simulink model "RRTMS_Activity_State"  (R2026a)
settings: Solver=FixedStepDiscrete  StopTime=10  FixedStep=1
settings Model: Creator=HP  LastModifiedBy=HP

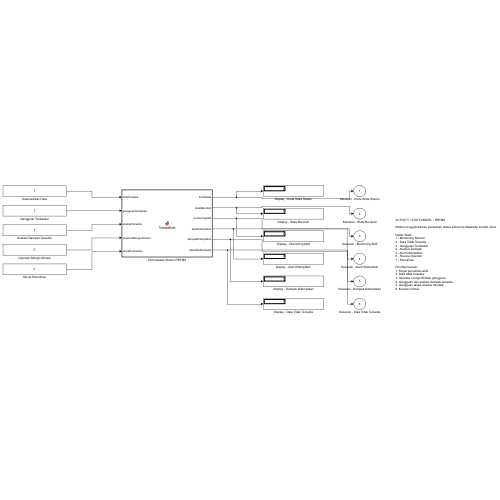
[thumbnail: Simulink's stored preview of the top-level diagram]
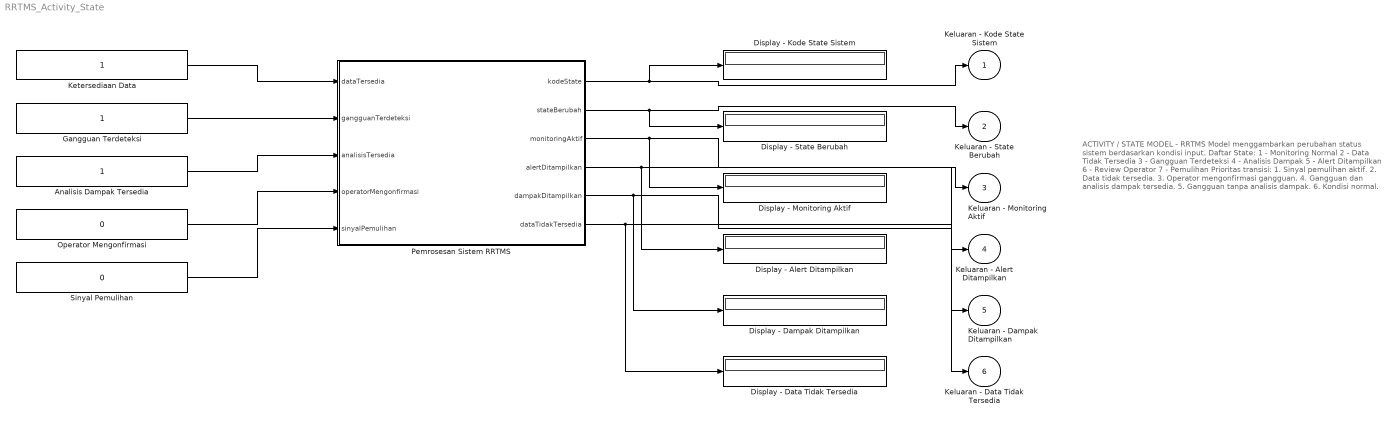
== system RRTMS_Activity_State ==
  note: ACTIVITY / STATE MODEL - RRTMS
      |
      | Model menggambarkan perubahan status sistem berdasarkan kondisi input.
      |
      | Daftar State:
      | 1 - Monitoring Normal
      | 2 - Data Tidak Tersedia
      | 3 - Gangguan Terdeteksi
      | 4 - Analisis Dampak
      | 5 - Alert Ditampilkan
      | 6 - Review Operator
      | 7 - Pemulihan
      |
      | Prioritas transisi:
      | 1. Sinyal pemulihan aktif.
      | 2. Data tidak tersedia.
      | 3. Operator mengonfirmasi gangguan.
      | 4. Gangguan dan analisis dampak tersedia.
      | 5. Gangguan tanpa analisis dampak.
      | 6. Kondisi normal.
  Analisis Dampak Tersedia : Constant
  Display - Alert Ditampilkan : Display
  Display - Dampak Ditampilkan : Display
  Display - Data Tidak Tersedia : Display
  Display - Kode State Sistem : Display
  Display - Monitoring Aktif : Display
  Display - State Berubah : Display
  Gangguan Terdeteksi : Constant
  Ketersediaan Data : Constant
  Operator Mengonfirmasi : Constant  Value=0
  Pemrosesan Sistem RRTMS : MATLAB Function  TreatAsAtomicUnit=on
  Sinyal Pemulihan : Constant  Value=0
  Keluaran - Kode State Sistem : Outport
  Keluaran - State Berubah : Outport  Port=2
  Keluaran - Monitoring Aktif : Outport  Port=3
  Keluaran - Alert Ditampilkan : Outport  Port=4
  Keluaran - Dampak Ditampilkan : Outport  Port=5
  Keluaran - Data Tidak Tersedia : Outport  Port=6
  wires:
  Ketersediaan Data/1 -> Pemrosesan Sistem RRTMS/1(dataTersedia)
  Gangguan Terdeteksi/1 -> Pemrosesan Sistem RRTMS/2(gangguanTerdeteksi)
  Analisis Dampak Tersedia/1 -> Pemrosesan Sistem RRTMS/3(analisisTersedia)
  Operator Mengonfirmasi/1 -> Pemrosesan Sistem RRTMS/4(operatorMengonfirmasi)
  Sinyal Pemulihan/1 -> Pemrosesan Sistem RRTMS/5(sinyalPemulihan)
  Pemrosesan Sistem RRTMS/1(kodeState) -> Display - Kode State Sistem/1, Keluaran - Kode State Sistem/1
  Pemrosesan Sistem RRTMS/2(stateBerubah) -> Display - State Berubah/1, Keluaran - State Berubah/1
  Pemrosesan Sistem RRTMS/3(monitoringAktif) -> Display - Monitoring Aktif/1, Keluaran - Monitoring Aktif/1
  Pemrosesan Sistem RRTMS/4(alertDitampilkan) -> Display - Alert Ditampilkan/1, Keluaran - Alert Ditampilkan/1
  Pemrosesan Sistem RRTMS/5(dampakDitampilkan) -> Display - Dampak Ditampilkan/1, Keluaran - Dampak Ditampilkan/1
  Pemrosesan Sistem RRTMS/6(dataTidakTersedia) -> Display - Data Tidak Tersedia/1, Keluaran - Data Tidak Tersedia/1

== matlab function RRTMS_Activity_State/Pemrosesan Sistem RRTMS ==
  data: dataTersedia input; kodeState output; gangguanTerdeteksi input; analisisTersedia input; operatorMengonfirmasi input; sinyalPemulihan input; stateBerubah output; monitoringAktif output; alertDitampilkan output; dampakDitampilkan output; dataTidakTersedia output
function [kodeState,stateBerubah,monitoringAktif,alertDitampilkan,dampakDitampilkan,dataTidakTersedia] = TransisiState(dataTersedia,gangguanTerdeteksi,analisisTersedia,operatorMengonfirmasi,sinyalPemulihan)
% State: 1=Monitoring, 2=Data unavailable, 3=Gangguan, 4=Analisis, 5=Alert, 6=Review, 7=Pemulihan
persistent state
if isempty(state)
    state = 1;
end
stateSebelumnya = state;
if sinyalPemulihan
    state = 7;
elseif ~dataTersedia
    state = 2;
elseif operatorMengonfirmasi && (stateSebelumnya == 3 || stateSebelumnya == 4 || stateSebelumnya == 5)
    state = 6;
elseif gangguanTerdeteksi
    if analisisTersedia
        if stateSebelumnya == 4
            state = 5;
        else
            state = 4;
        end
    else
        state = 3;
    end
else
    state = 1;
end
kodeState = state;
stateBerubah = (state ~= stateSebelumnya);
monitoringAktif = dataTersedia && (state ~= 7);
alertDitampilkan = (state == 3 || state == 4 || state == 5);
dampakDitampilkan = (state == 4 || state == 5);
dataTidakTersedia = (state == 2);
end
